simulink model "Twin_Builder"  (R2026a)
settings: Solver=VariableStepAuto  StopTime=simTime  FixedStep=Ts/60  RelTol=1e-2
values from neighbouring files (symbols this model uses):
  ac = log(9)/tr    [Run_Twin.m]
  as = 0.08 * ac    [Run_Twin.m]
  ath = 0.25 * as    [Run_Twin.m]
  B = 0.00001    (= 1e-05)    [Run_Twin.m]
  BEMFD_FEA_PerHz = InterpFEA_Data_ForSimulink(FEA_Data.BackEMFD_perHz, IS_FEA, IEA_FEA, IS_Interp, IEA_Interp)    [Run_Twin.m]
  BEMFQ_FEA_PerHz = InterpFEA_Data_ForSimulink(FEA_Data.BackEMFQ_perHz, IS_FEA, IEA_FEA, IS_Interp, IEA_Interp)    [Run_Twin.m]
  CondLoss_Inv = zeros([length(IS_Interp), size(FEA_Data.ConductionLoss, [2 3] ) ])    [Run_Twin.m]
  CopperLoss_FEA = InterpFEA_Data_ForSimulink(FEA_Data.CopperLosses, IS_FEA, IEA_FEA, IS_Interp, IEA_Interp)    [Run_Twin.m]
  DriveMethod = 1    [Run_Twin.m]
  EnvTorque_FW = interp1(Speed_full, Env_full, Speed_Vec, 'pchip', 'extrap')    [Run_Twin.m]
  f_sw = 10e3    (= 10000)    [Run_Twin.m]
  FEA_Data = LoadData.(FieldData{1})    [Run_Twin.m]
  FILTER_COEFF = 0.23    [Run_Twin.m]
  FluxD_FEA = InterpFEA_Data_ForSimulink(FEA_Data.FluxD, IS_FEA, IEA_FEA, IS_Interp, IEA_Interp)    [Run_Twin.m]
  FluxQ_FEA = InterpFEA_Data_ForSimulink(FEA_Data.FluxQ, IS_FEA, IEA_FEA, IS_Interp, IEA_Interp)    [Run_Twin.m]
  FrictLoss_FEA = squeeze( FEA_Data.FrictLosses(1,1,:) )    [Run_Twin.m]
  GateLoss_Inv = zeros([length(IS_Interp), size(FEA_Data.ConductionLoss, [2 3] ) ])    [Run_Twin.m]
  IDcore_FEA = InterpFEA_Data_ForSimulink(FEA_Data.IDc, IS_FEA, IEA_FEA, IS_Interp, IEA_Interp)    [Run_Twin.m]
  IEA_FEA = IEA_Interp    [Run_Twin.m]
  IQcore_FEA = InterpFEA_Data_ForSimulink(FEA_Data.IQc, IS_FEA, IEA_FEA, IS_Interp, IEA_Interp)    [Run_Twin.m]
  IronLoss_FEA = InterpFEA_Data_ForSimulink(FEA_Data.IronLosses,   IS_FEA, IEA_FEA, IS_Interp, IEA_Interp)    [Run_Twin.m]
  Is_Amp = 40    [Run_Twin.m]
  IS_FEA = IS_Interp    [Run_Twin.m]
  J = FEA_Data.Jinertia    [Run_Twin.m]
  J_Control = FEA_Data.Jinertia    [Run_Twin.m]
  LD_FEA = InterpFEA_Data_ForSimulink(FEA_Data.LD, IS_FEA, IEA_FEA, IS_Interp, IEA_Interp)    [Run_Twin.m]
  LD_Single = mean(LD_FEA, 'all')    [Run_Twin.m]
  LQ_FEA = InterpFEA_Data_ForSimulink(FEA_Data.LQ, IS_FEA, IEA_FEA, IS_Interp, IEA_Interp)    [Run_Twin.m]
  LQ_Single = mean(LQ_FEA, 'all')    [Run_Twin.m]
  MagnetLoss_FEA = InterpFEA_Data_ForSimulink(FEA_Data.MagnetLosses, IS_FEA, IEA_FEA, IS_Interp, IEA_Interp)    [Run_Twin.m]
  MaxSpeed = max(Speed_Vec)    [Run_Twin.m]
  MaxTe = max(Torque_FEA, [], 'all')    [Run_Twin.m]
  ModStrategy = 1    [Run_Twin.m]
  PMFlux_FEA = interp1(IS_FEA, squeeze( FEA_Data.FluxD(:,IEA_FEA == 90, :) ), IS_Interp, 'pchip' )    [Run_Twin.m]
  PMFlux_Single = mean( PMFlux_FEA, 'all' )    [Run_Twin.m]
  PMT_ID = round( F_ID(PMT_grid, Speed_grid), 2)    [Run_Twin.m]
  PMT_IQ = round( F_IQ(PMT_grid, Speed_grid), 2)    [Run_Twin.m]
  PMT_Vec = linspace(0,   100,   InterpSamples)    [Run_Twin.m]
  PolePair = FEA_Data.Poles / 2    [Run_Twin.m]
  PPR = 1024    [Run_Twin.m]
  ProxiLoss_FEA = InterpFEA_Data_ForSimulink(FEA_Data.ProxiLosses,  IS_FEA, IEA_FEA, IS_Interp, IEA_Interp)    [Run_Twin.m]
  Rcore_FEA = InterpFEA_Data_ForSimulink(FEA_Data.Rcore, IS_FEA, IEA_FEA, IS_Interp, IEA_Interp)    [Run_Twin.m]
  RDC = squeeze( Rseries_FEA(1,1,1) )    [Run_Twin.m]
  RefSpeed = [50, 400, 250, 500, 400]    [Run_Twin.m]
  RefTheta = [50, 0, 140, 300, -50]    [Run_Twin.m]
  Rseries_FEA = InterpFEA_Data_ForSimulink(FEA_Data.Rs,    IS_FEA, IEA_FEA, IS_Interp, IEA_Interp)    [Run_Twin.m]
  ShafthLoad = [10, 25, 3, 8, 10]    [Run_Twin.m]
  simTime = mechThetaTarget / wMechTarget    [Run_Twin.m]
  Speed_FEA = FEA_Data.Speed_vec    [Run_Twin.m]
  Speed_Vec = linspace(min(Speed_full), max(Speed_full), InterpSamples)    [Run_Twin.m]
  speedTarget = 200    [Run_Twin.m]
  SR_FEA = FEA_Data.SynchAngle    [Run_Twin.m]
  SwitchLoss_Inv = zeros([length(IS_Interp), size(FEA_Data.ConductionLoss, [2 3] ) ])    [Run_Twin.m]
  Tdt = 0.3 * 1e-6    (= 3e-07)    [Run_Twin.m]
  Throttle = 45    [Run_Twin.m]
  Times = [0, 0.2, 0.4, 0.6, 0.8] * simTime    [Run_Twin.m]
  Torque_FEA = InterpFEA_Data_ForSimulink(FEA_Data.TorqueFEA, IS_FEA, IEA_FEA, IS_Interp, IEA_Interp)    [Run_Twin.m]
  Ts = 1/f_sw    (= 0.0001)    [Run_Twin.m]
  Ts_Sp = 2 * Ts    (= 0.0002)    [Run_Twin.m]
  Vdc = 56    [Run_Twin.m]
  Vs_pu = 0.98    [Run_Twin.m]
  WindageLoss_FEA = squeeze( FEA_Data.WindLosses(1,1,:) )    [Run_Twin.m]
undefined symbols (not defined in the file or in its folder): DiscIntNeverNeededParam, feNom, mf, OverMod, PMT_Speed, SimData, Tables
libraries: simulink x14, ee_lib x11, simulink_extras x7, eeTransforms x6, fl_lib x6, eeGeneralControl x4, spsMeanLib x2, dspxfrm3 x1
(part 1 of 3)
settings Model: Creator=antho  LastModifiedBy=antho
settings SolverCC: ZeroCrossAlgorithm=Adaptive
settings DebuggingCC: ArtificialAlgebraicLoopMsg=none  MaskedZcDiagnostic=none  IgnoredZcDiagnostic=none
settings SimscapeCC: SimscapeNominalValues="[{\"value\":\"1\",\"unit\":\"A\"},{\"value\":\"1\",\"unit\":\"bar\"},{\"value\":\"1\",\"unit\":\"cm^2\"},{\"value\":\"1\",\"unit\":\"cm^3/s\"},{\"value\":\"1\",\"unit\":\"kJ/kg\"},{\"value\":\"1\",\"unit\":\"kW\"},{\"value\":\"1\",\"unit\":\"l\"},{\"value\":\"1\",\"unit\":\"N\"},{\"value\":\"1\",\"unit\":\"N*m\"},{\"value\":\"1\",\"unit\":\"V\"}]"  SimscapeLogType=none  SimscapeLogDataHistory=5000.0

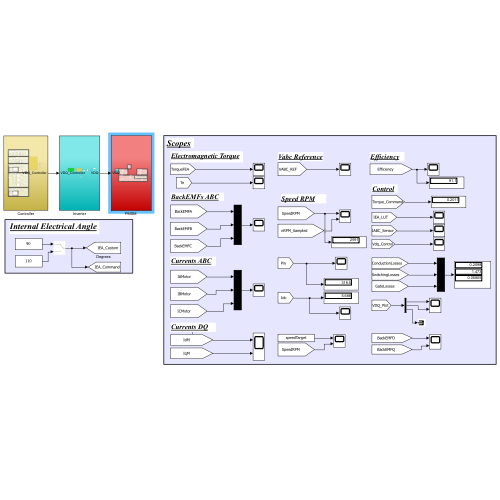
[thumbnail: Simulink's stored preview of the top-level diagram]
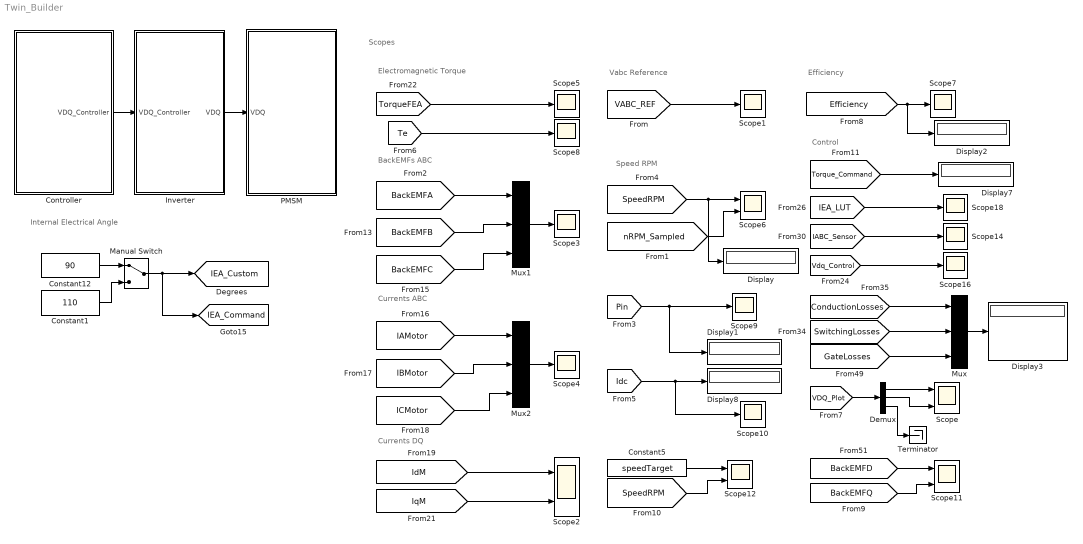
== system Twin_Builder ==
  note: Currents ABC
  note: BackEMFs ABC
  note: Scopes
  note: Electromagnetic Torque
  note: Currents DQ
  note: Vabc Reference
  note: Speed RPM
  note: Internal Electrical Angle
  note: Efficiency
  note: Control
  Constant1 : Constant  Value=110  VectorParams1D=off  SampleTime=0
  Constant12 : Constant  Value=90  VectorParams1D=off  SampleTime=0
  Constant5 : Constant  Value=speedTarget  SampleTime=Ts
  Controller : Subsystem
  Demux : Demux  Outputs=3
  Display{,1..3,7..8} (6 alike) : Display
  Inverter : Subsystem
  Manual Switch : ManualSwitch
  Mux : Mux  Inputs=3
  Mux1 : Mux  Inputs=3
  Mux2 : Mux  Inputs=3
  "PMSM " : Subsystem
  Scope{,2,6,11..12} (5 alike) : Scope  NumInputPorts=2
      Scope settings: ActiveDisplayYMinimum=-43.33518  ActiveDisplayYMaximum=40.81845
      Scope11 settings: ActiveDisplayYMinimum=-5.31808  ActiveDisplayYMaximum=1.44392  DataLoggingVariableName=ScopeData2
      Scope12 settings: ActiveDisplayYMinimum=1475.9301024865783  ActiveDisplayYMaximum=1516.335592593025  DataLoggingVariableName=ScopeData22
      Scope2 settings: ActiveDisplayYMinimum=-5.9549540447298286  ActiveDisplayYMaximum=6.9473157264243515  DataLoggingVariableName=ScopeData7
      Scope6 settings: ActiveDisplayYMinimum=-188.56958986761623  ActiveDisplayYMaximum=1697.1263088085464
  Scope{1,3..5,7..10,14,16,18} (11 alike) : Scope
      Scope1 settings: ActiveDisplayYMinimum=-0.12499999999999997  ActiveDisplayYMaximum=1.125
      Scope10 settings: ActiveDisplayYMinimum=-10.699535134143511  ActiveDisplayYMaximum=61.951701868549058
      Scope14 settings: ActiveDisplayYMinimum=-35.97658  ActiveDisplayYMaximum=53.42367
      Scope16 settings: ActiveDisplayYMinimum=-13.11859  ActiveDisplayYMaximum=37.37662  DataLoggingVariableName=ScopeData5
      Scope18 settings: ActiveDisplayYMinimum=26.32642  ActiveDisplayYMaximum=197.07481
      Scope3 settings: ActiveDisplayYMinimum=-28.0068607396772  ActiveDisplayYMaximum=28.009786105867875  DataLoggingVariableName=ScopeData25
      Scope4 settings: ActiveDisplayYMinimum=-10.513567775174659  ActiveDisplayYMaximum=10.513016915714479  DataLoggingVariableName=ScopeData3
      Scope5 settings: ActiveDisplayYMinimum=0.36126733092148122  ActiveDisplayYMaximum=0.991709204534436  DataLoggingVariableName=ScopeData2
      Scope7 settings: ActiveDisplayYMinimum=90.703551699385159  ActiveDisplayYMaximum=92.220982491183165
      Scope8 settings: ActiveDisplayYMinimum=-8.4790158509726883  ActiveDisplayYMaximum=35.221572331501939  DataLoggingVariableName=ScopeData3
      Scope9 settings: ActiveDisplayYMinimum=-526.14083348977579  ActiveDisplayYMaximum=1930.1579846280983
  Terminator : Terminator
  tag scope: IEA_Command=global, IEA_Custom=global
  wires:
  [BackEMFB] -> Mux1/2
  [BackEMFA] -> Mux1/1
  [IqM] -> Scope2/2
  [BackEMFC] -> Mux1/3
  [IBMotor] -> Mux2/2
  Mux1/1 -> Scope3/1
  [ICMotor] -> Mux2/3
  Mux2/1 -> Scope4/1
  [IAMotor] -> Mux2/1
  [TorqueFEA] -> Scope5/1
  [IdM] -> Scope2/1
  [VABC_REF] -> Scope1/1
  [SpeedRPM] -> Scope6/1, Display/1
  Inverter/1(VDQ) -> "PMSM "/1(VDQ)
  [Te] -> Scope8/1
  [Efficiency] -> Display2/1, Scope7/1
  Controller/1(VDQ_Controller) -> Inverter/1(VDQ_Controller)
  [Torque_Command] -> Display7/1
  Constant12/1 -> Manual Switch/1
  Manual Switch/1 -> [IEA_Command], [IEA_Custom]
  Constant1/1 -> Manual Switch/2
  [Vdq_Control] -> Scope16/1
  [IEA_LUT] -> Scope18/1
  [IABC_Sensor] -> Scope14/1
  [nRPM_Sampled] -> Scope6/2
  [Pin] -> Display1/1, Scope9/1
  [GateLosses] -> Mux/3
  [SwitchingLosses] -> Mux/2
  [ConductionLosses] -> Mux/1
  Mux/1 -> Display3/1
  [Idc] -> Scope10/1, Display8/1
  Demux/3 -> Terminator/1
  Demux/2 -> Scope/2
  Demux/1 -> Scope/1
  [VDQ_Plot] -> Demux/1
  [BackEMFD] -> Scope11/1
  [BackEMFQ] -> Scope11/2
  Constant5/1 -> Scope12/1
  [SpeedRPM] -> Scope12/2

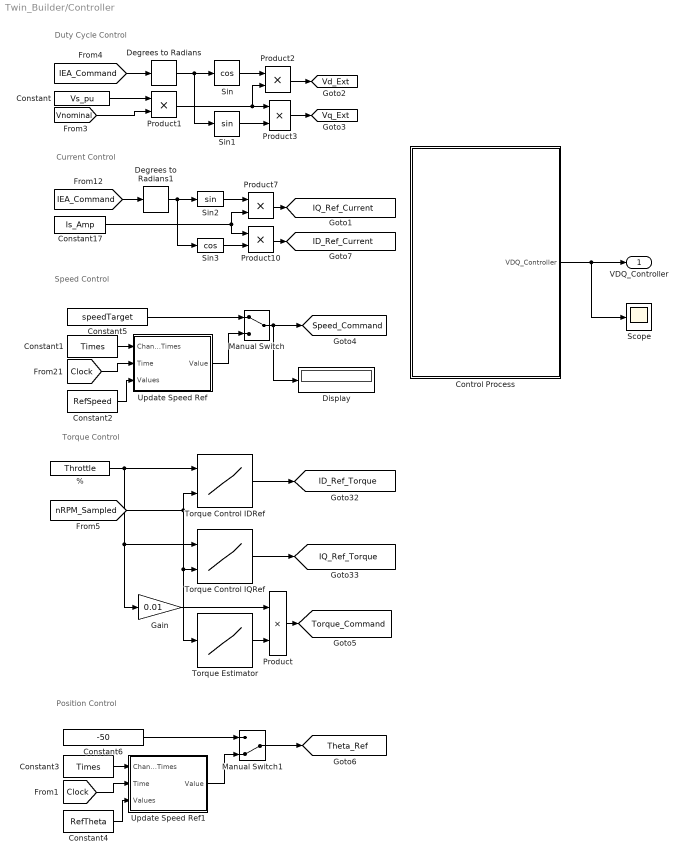
== system Twin_Builder/Controller ==
  note: Duty Cycle Control
  note: Speed Control
  note: Current Control
  note: Torque Control
  note: Position Control
  % : Constant  Value=Throttle  VectorParams1D=off  SampleTime=0
  Constant : Constant  Value=Vs_pu  SampleTime=0
  Constant1 : Constant  Value=Times
  Constant17 : Constant  Value=Is_Amp  SampleTime=0
  Constant2 : Constant  Value=RefSpeed
  Constant3 : Constant  Value=Times
  Constant4 : Constant  Value=RefTheta
  Constant5 : Constant  Value=speedTarget  SampleTime=Ts
  Constant6 : Constant  Value=-50  SampleTime=Ts
  Control Process : Subsystem
  Degrees to Radians : simulink_extras/Transformations/Degrees to Radians
  Degrees to Radians1 : simulink_extras/Transformations/Degrees to Radians
  Display : Display
  Gain : Gain  Gain=0.01
  Manual Switch : ManualSwitch
  Manual Switch1 : ManualSwitch  CurrentSetting=0
  Product{,1..3,7,10} (6 alike) : Product
  Scope : Scope
      settings: ActiveDisplayYMinimum=-9.29519  ActiveDisplayYMaximum=32.08868  DataLoggingVariableName=ScopeData2
  Sin : Trigonometry  Operator=cos
  Sin1 : Trigonometry
  Sin2 : Trigonometry
  Sin3 : Trigonometry  Operator=cos
  Torque Control IDRef : Lookup_n-D  BreakpointsForDimension1=PMT_Vec  BreakpointsForDimension2=Speed_Vec  Table=PMT_ID  InternalRulePriority=Speed  RndMeth=Simplest
      settings: InputPortMap=u0,u1
  Torque Control IQRef : Lookup_n-D  BreakpointsForDimension1=PMT_Vec  BreakpointsForDimension2=Speed_Vec  Table=PMT_IQ  InternalRulePriority=Speed  RndMeth=Simplest
      settings: InputPortMap=u0,u1
  Torque Estimator : Lookup_n-D  NumberOfTableDimensions=1  BreakpointsForDimension1=Speed_Vec  BreakpointsForDimension2=PMT_Speed(1,:)  Table=EnvTorque_FW  InternalRulePriority=Speed  RndMeth=Simplest
  Update Speed Ref : MATLAB Function  TreatAsAtomicUnit=on
  Update Speed Ref1 : MATLAB Function  TreatAsAtomicUnit=on
  VDQ_Controller : Outport
  tag scope: ID_Ref_Current=global, ID_Ref_Torque=global, IQ_Ref_Current=global, IQ_Ref_Torque=global, Speed_Command=global, Theta_Ref=global, Torque_Command=global, Vd_Ext=global, Vq_Ext=global
  wires:
  Product2/1 -> [Vd_Ext]
  Product3/1 -> [Vq_Ext]
  Product1/1 -> Product2/2, Product3/1
  Degrees to Radians/1 -> Sin/1, Sin1/1
  Sin1/1 -> Product3/2
  Sin/1 -> Product2/1
  [IEA_Command] -> Degrees to Radians/1
  Constant/1 -> Product1/1
  [Vnominal] -> Product1/2
  Product7/1 -> [IQ_Ref_Current]
  Degrees to Radians1/1 -> Sin3/1, Sin2/1
  Sin2/1 -> Product7/1
  Product10/1 -> [ID_Ref_Current]
  [IEA_Command] -> Degrees to Radians1/1
  Constant17/1 -> Product10/1, Product7/2
  Sin3/1 -> Product10/2
  %/1 -> Torque Control IDRef/1, Torque Control IQRef/1, Gain/1
  Torque Control IQRef/1 -> [IQ_Ref_Torque]
  Torque Control IDRef/1 -> [ID_Ref_Torque]
  [nRPM_Sampled] -> Torque Estimator/1, Torque Control IQRef/2, Torque Control IDRef/2
  Product/1 -> [Torque_Command]
  Torque Estimator/1 -> Product/2
  Gain/1 -> Product/1
  Update Speed Ref/1(Value) -> Manual Switch/2
  Constant2/1 -> Update Speed Ref/3(Values)
  Constant1/1 -> Update Speed Ref/1(ChangeTimes)
  [Clock] -> Update Speed Ref/2(Time)
  Constant5/1 -> Manual Switch/1
  Manual Switch/1 -> Display/1, [Speed_Command]
  Control Process/1(VDQ_Controller) -> VDQ_Controller/1, Scope/1
  Constant3/1 -> Update Speed Ref1/1(ChangeTimes)
  Update Speed Ref1/1(Value) -> Manual Switch1/2
  [Clock] -> Update Speed Ref1/2(Time)
  Constant4/1 -> Update Speed Ref1/3(Values)
  Manual Switch1/1 -> [Theta_Ref]
  Constant6/1 -> Manual Switch1/1

== system Twin_Builder/Inverter ==
  VDQ_Controller : Inport
  Create VRef : Subsystem
  MCU Delay : Delay  Commented=on  DelayLength=1  SampleTime=1.5*Ts
  Manual Switch : ManualSwitch  CurrentSetting=0
  PowerSwitches : Subsystem
  VDQ : Outport
  tag scope: VDQ_Plot=global
  wires:
  VDQ_Controller/1 -> Create VRef/1(VDQ_Controller)
  Create VRef/1(Vabc_Ref) -> PowerSwitches/1(Vabc_Ref)
  PowerSwitches/1(Vdq0) -> Manual Switch/1
  Manual Switch/1 -> [VDQ_Plot], VDQ/1
  [Vdq_Control] -> Manual Switch/2

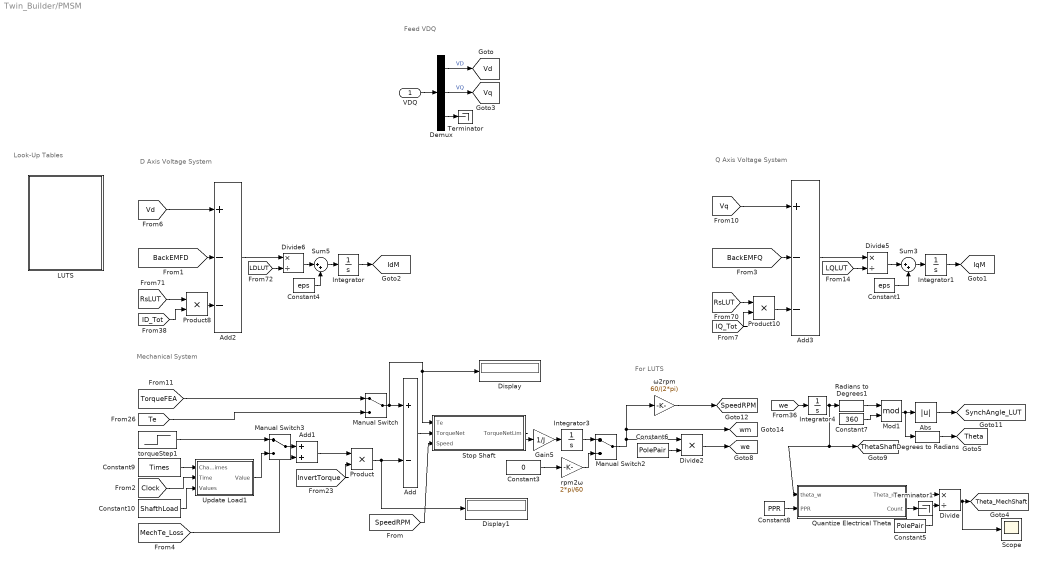
== system Twin_Builder/PMSM  ==
  note: Q Axis Voltage System
  note: D Axis Voltage System
  note: Feed VDQ
  note: Look-Up Tables
  note: Mechanical System
  note: For LUTS
  VDQ : Inport
  Abs : Abs  SaturateOnIntegerOverflow=off
  Add : Sum  Inputs=+-
  Add1 : Sum
  Add2 : Sum  Inputs=+--
  Add3 : Sum  Inputs=+--
  Constant1 : Constant  Value=eps  SampleTime=0
  Constant10 : Constant  Value=ShafthLoad
  Constant3 : Constant  Value=0  SampleTime=0
  Constant4 : Constant  Value=eps  SampleTime=0
  Constant5 : Constant  Value=PolePair
  Constant6 : Constant  Value=PolePair
  Constant7 : Constant  Value=360
  Constant8 : Constant  Value=PPR
  Constant9 : Constant  Value=Times
  Degrees to Radians : simulink_extras/Transformations/Degrees to Radians
  Demux : Demux  Outputs=3
  Display : Display
  Display1 : Display
  Divide : Product  Inputs=*/
  Divide2 : Product  Inputs=**
  Divide5 : Product  Inputs=*/
  Divide6 : Product  Inputs=*/
  Gain5 : Gain  Gain=1/J
  Integrator{,1,3..4} (4 alike) : Integrator
  LUTS : Subsystem
  Manual Switch : ManualSwitch
  Manual Switch2 : ManualSwitch
  Manual Switch3 : ManualSwitch
  Mod1 : Math  Operator=mod
  Product : Product
  Product10 : Product
  Product8 : Product
  "Quantize Electrical Theta " : MATLAB Function  TreatAsAtomicUnit=on
  Radians to Degrees1 : simulink_extras/Transformations/Radians to Degrees
  Scope : Scope
      settings: ActiveDisplayYMinimum=6.6141363545978225  ActiveDisplayYMaximum=6.6434972553948457  DataLoggingVariableName=ScopeData31
  Stop Shaft : MATLAB Function  TreatAsAtomicUnit=on
  Sum3 : Sum  Inputs=|++
  Sum5 : Sum  Inputs=|++
  Terminator : Terminator
  Terminator1 : Terminator
  Update Load1 : MATLAB Function  TreatAsAtomicUnit=on
  rpm2ω : Gain  Gain=2*pi/60
  torqueStep1 : Step  Time=0  FinalValue=mechLoad  SampleTime=0
  ω2rpm : Gain  Gain=60/(2*pi)
  tag scope: IdM=global, IqM=global, SpeedRPM=global, SynchAngle_LUT=global, Theta=global, ThetaShaft=global, Theta_MechShaft=global, Vd=global, Vq=global, we=global, wm=global
  wires:
  [Vd] -> Add2/1
  [BackEMFQ] -> Add3/2
  Constant4/1 -> Sum5/2
  [LQLUT] -> Divide5/2
  [LDLUT] -> Divide6/2
  Divide6/1 -> Sum5/1
  Product10/1 -> Add3/3
  [IQ_Tot] -> Product10/2
  Product8/1 -> Add2/3
  Sum3/1 -> Integrator1/1
  [BackEMFD] -> Add2/2
  [ID_Tot] -> Product8/2
  Constant1/1 -> Sum3/2
  [RsLUT] -> Product8/1
  Sum5/1 -> Integrator/1
  [Vq] -> Add3/1
  Divide5/1 -> Sum3/1
  [RsLUT] -> Product10/1
  Add3/1 -> Divide5/1
  Add2/1 -> Divide6/1
  Demux/3 -> Terminator/1
  VDQ/1 -> Demux/1
  Demux/1 -> [Vd]  "VD"
  Demux/2 -> [Vq]  "VQ"
  Integrator/1 -> [IdM]
  Integrator1/1 -> [IqM]
  [Te] -> Manual Switch/2
  Gain5/1 -> Integrator3/1
  [TorqueFEA] -> Manual Switch/1
  Integrator4/1 -> "Quantize Electrical Theta "/1(theta_w), [ThetaShaft], Radians to Degrees1/1
  Constant7/1 -> Mod1/2
  Abs/1 -> [SynchAngle_LUT]
  ω2rpm/1 -> [SpeedRPM]
  Divide2/1 -> [we]
  Constant6/1 -> Divide2/2
  [we] -> Integrator4/1
  Radians to Degrees1/1 -> Mod1/1
  Mod1/1 -> Degrees to Radians/1, Abs/1
  Degrees to Radians/1 -> [Theta]
  [SpeedRPM] -> Stop Shaft/3(Speed)
  Add/1 -> Stop Shaft/2(TorqueNet)
  Stop Shaft/1(TorqueNetLim) -> Gain5/1
  Manual Switch/1 -> Display/1, Stop Shaft/1(Te), Add/1
  Integrator3/1 -> Manual Switch2/1
  Manual Switch2/1 -> Divide2/1, [wm], ω2rpm/1
  rpm2ω/1 -> Manual Switch2/2
  Constant3/1 -> rpm2ω/1
  Constant8/1 -> "Quantize Electrical Theta "/2(PPR)
  "Quantize Electrical Theta "/2(Count) -> Terminator1/1
  Constant5/1 -> Divide/2
  "Quantize Electrical Theta "/1(Theta_mcu) -> Divide/1
  Divide/1 -> Scope/1, [Theta_MechShaft]
  Constant9/1 -> Update Load1/1(ChangeTimes)
  Constant10/1 -> Update Load1/3(Values)
  [MechTe_Loss] -> Add1/2
  [Clock] -> Update Load1/2(Time)
  torqueStep1/1 -> Manual Switch3/1
  Update Load1/1(Value) -> Manual Switch3/2
  Manual Switch3/1 -> Add1/1
  [InvertTorque] -> Product/2
  Add1/1 -> Product/1
  Product/1 -> Display1/1, Add/2

== system Twin_Builder/Controller/Control Process ==
  Add2 : Sum
  Constant : Constant  Value=0
  Display2 : Display
  IDQ References from Speed Controller : Subsystem
  IDQ _Reference : Subsystem
  Mux : Mux  Inputs=2
  Speed Reference from Position Controller : Subsystem
  VDQ Reference from Current Controller Fundamental : Subsystem
  VDQ Reference from Voltage Controller : Subsystem
  Voltage Saturation : Subsystem
  VDQ_Controller : Outport
  wires:
  [ID_Ref] -> VDQ Reference from Current Controller Fundamental/1(ID_Ref)
  VDQ Reference from Current Controller Fundamental/1(VDQ_Current) -> Add2/1
  [Speed_Ref] -> IDQ References from Speed Controller/1(SpeedRef)
  [Vd_Ext] -> VDQ Reference from Voltage Controller/1(Vd_Ext)
  [Vq_Ext] -> VDQ Reference from Voltage Controller/2(Vq_Ext)
  VDQ Reference from Voltage Controller/1(VDQ_Voltage) -> Add2/2
  [IQ_Ref] -> Display2/1, VDQ Reference from Current Controller Fundamental/2("IQ_Ref ")
  [Theta_Ref] -> Speed Reference from Position Controller/1(Theta_Ref)
  Add2/1 -> Mux/1
  Constant/1 -> Mux/2
  Mux/1 -> VDQ_Controller/1

== system Twin_Builder/Inverter/Create VRef ==
  note: Vabc_Ref Generation
  VDQ_Controller : Inport
  Add2 : Sum
  Constant : Constant  Value=OverMod  SampleTime=0
  Determine Common Mode Signal : Subsystem
  Divide : Product  Inputs=**/
  Finalize References : Subsystem
  Inverse Park Transform : eeTransforms/Inverse Park Transform  AxisAlignment=D-axis  PowerInvariant=off
      settings: LibrarySourceBlock=|
      | ee_sl_lib/Mathematical
      | Transforms/Inverse
      | Park Transform
  Park Transform : eeTransforms/Park Transform  AxisAlignment=D-axis  PowerInvariant=off
      settings: LibrarySourceBlock=|
      | ee_sl_lib/Mathematical
      | Transforms/Park Transform
  Product : Product
  Product1 : Product
  Sample References : MATLAB Function  TreatAsAtomicUnit=on
  Scope : Scope
      settings: ActiveDisplayYMinimum=-0.125  ActiveDisplayYMaximum=1.125  DataLoggingVariableName=ScopeData4
  Vabc_Ref : Outport
  tag scope: VABC_REF=global, VDQ=global, Vabc_SPWM=global, Vdq_Control=global
  wires:
  [Theta_Sampled] -> Inverse Park Transform/2
  [CommonMode] -> Add2/2
  [Vnominal] -> Divide/3
  Constant/1 -> Divide/2
  [Overmod] -> Product/2
  [Vnominal] -> Product1/2
  Product1/1 -> [Vdq_Control]
  [Theta_Sampled] -> Park Transform/2
  Inverse Park Transform/1 -> Divide/1
  Add2/1 -> Product/1
  VDQ_Controller/1 -> [VDQ], Inverse Park Transform/1
  Divide/1 -> [Vabc_SPWM], Add2/1
  Finalize References/1(Vabc_Ref_Final) -> [VABC_REF], Scope/1, Vabc_Ref/1
  [Carrier] -> Sample References/2(TriSignal)
  Sample References/1(SampledSignals) -> Park Transform/1, Finalize References/1(Vabc_Ref)
  Product/1 -> Sample References/1(Signal)
  Park Transform/1 -> Product1/1

== system Twin_Builder/Inverter/PowerSwitches ==
  note: Inverter
  Vabc_Ref : Inport
  0.5 Ts PWM delay : Delay  DelayLength=1  SampleTime=Ts/2
  Add1 : Sum  Inputs=+-
  Cast To Boolean : DataTypeConversion  Commented=on  OutDataTypeStr=double  SaturateOnIntegerOverflow=off  RndMeth=Floor
  Cast To Boolean1 : DataTypeConversion  Commented=on  OutDataTypeStr=double  SaturateOnIntegerOverflow=off  RndMeth=Floor
  Cast To Boolean2 : DataTypeConversion  Commented=on  OutDataTypeStr=double  SaturateOnIntegerOverflow=off  RndMeth=Floor
  Cast To Boolean3 : DataTypeConversion  Commented=on  OutDataTypeStr=boolean  SaturateOnIntegerOverflow=off  RndMeth=Floor
  Cast To Boolean4 : DataTypeConversion  Commented=on  OutDataTypeStr=boolean  SaturateOnIntegerOverflow=off  RndMeth=Floor
  Cast To Boolean5 : DataTypeConversion  Commented=on  OutDataTypeStr=boolean  SaturateOnIntegerOverflow=off  RndMeth=Floor
  Constant2 : Constant  Value=Vdc  SampleTime=0
  Gain2 : Gain  Gain=1/3  RndMeth=Round  OutDataTypeStr=Inherit: Same as input
  Park Transform : eeTransforms/Park Transform  AxisAlignment=D-axis  PowerInvariant=off
      settings: LibrarySourceBlock=|
      | ee_sl_lib/Mathematical
      | Transforms/Park Transform
  Product1 : Product
  Relational Operator3 : RelationalOperator  OutDataTypeStr=boolean  RndMeth=Simplest  InputSameDT=off
  Scope1 : Scope
      settings: ActiveDisplayYMinimum=-40  ActiveDisplayYMaximum=40  DataLoggingVariableName=ScopeData2
  Sum of Elements : Sum  Inputs=+
  Transport Delay1 : TransportDelay  Commented=on  DelayTime=Tdt  TransDelayFeedthrough=on
  Transport Delay2 : TransportDelay  Commented=on  DelayTime=Tdt
  Transport Delay3 : TransportDelay  Commented=on  DelayTime=Tdt
  Vdq0 : Outport
  tag scope: VabcInv=global
  wires:
  Cast To Boolean1/1 -> Transport Delay2/1
  Cast To Boolean/1 -> Transport Delay1/1
  Transport Delay3/1 -> Cast To Boolean5/1
  Transport Delay2/1 -> Cast To Boolean4/1
  Transport Delay1/1 -> Cast To Boolean3/1
  Cast To Boolean2/1 -> Transport Delay3/1
  Vabc_Ref/1 -> 0.5 Ts PWM delay/1
  [Carrier] -> Relational Operator3/2
  Constant2/1 -> Product1/2
  Sum of Elements/1 -> Gain2/1
  Gain2/1 -> Add1/2
  Product1/1 -> Sum of Elements/1, Add1/1
  Add1/1 -> Park Transform/1, [VabcInv], Scope1/1
  [Theta] -> Park Transform/2
  Park Transform/1 -> Vdq0/1
  Relational Operator3/1 -> Product1/1
  0.5 Ts PWM delay/1 -> Relational Operator3/1

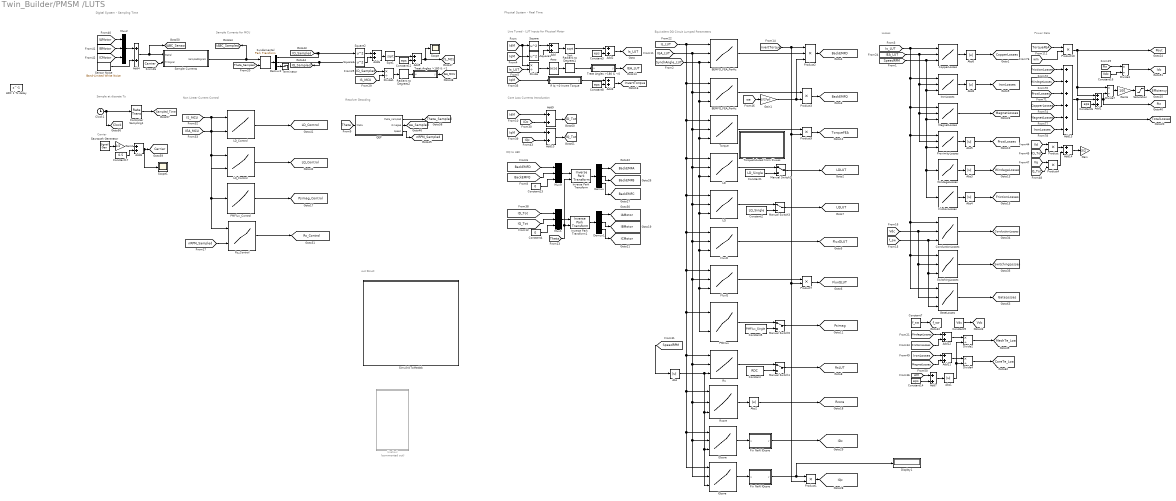
== system Twin_Builder/PMSM /LUTS ==
  note: out Struct
  note: Power Data
  note: Losses
  note: Equivalent DQ Circuit Lumped Parameters
  note: DQ to ABC
  note: Live Tuned - LUT Inputs for Physical Motor
  note: Physical System - Real Time
  note: Sample at discrete Ts
  note: Sample Currents for MCU
  note: Resolver Decoding
  note: Non Linear Current Control
  note: Digital System - Sampling Time
  note: Carrier
  note: Core Loss Currents Introduction
  ADC 1 Ts delay : Delay  DelayLength=1  SampleTime=Ts
  Abs{,1..6,8} (8 alike) : Abs  SaturateOnIntegerOverflow=off
  Acos : Trigonometry  Operator=acos  OutputSignalType=real
  Add{,2..12,14} (13 alike) : Sum
  Add1 : Sum  Inputs=+++
  Add13 : Sum  Inputs=++++++
  BEMFD_FEA_PerHz : Lookup_n-D  NumberOfTableDimensions=3  BreakpointsForDimension1=IS_FEA  BreakpointsForDimension2=IEA_FEA  BreakpointsForDimension3=SR_FEA  Table=BEMFD_FEA_PerHz  InternalRulePriority=Speed  RndMeth=Simplest
      settings: InputPortMap=u0,u1,u2
  BEMFQ_FEA_PerHz : Lookup_n-D  NumberOfTableDimensions=3  BreakpointsForDimension1=IS_FEA  BreakpointsForDimension2=IEA_FEA  BreakpointsForDimension3=SR_FEA  Table=BEMFQ_FEA_PerHz  InternalRulePriority=Speed  RndMeth=Simplest
      settings: InputPortMap=u0,u1,u2
  Clock1 : Clock
  ConductionLosses : Lookup_n-D  NumberOfTableDimensions=3  BreakpointsForDimension1=IS_FEA  BreakpointsForDimension2=FEA_Data.Vds_Vec  BreakpointsForDimension3=FEA_Data.fsw_Vec  BreakpointsForDimension4=FEA_Data.fsw_Vec  Table=CondLoss_Inv  InternalRulePriority=Speed  RndMeth=Simplest
      settings: InputPortMap=u0,u1,u2
  Constant : Constant  Value=RDC  SampleTime=0
  Constant1 : Constant  Value=LD_Single  SampleTime=0
  Constant{3,6,8,12} (4 alike) : Constant  Value=eps  SampleTime=0
  Constant13 : Constant  Value=0  SampleTime=0
  Constant14 : Constant  Value=eps
  Constant16 : Constant  Value=Vdc  SampleTime=0
  Constant17 : Constant  Value=0.5  SampleTime=0
  Constant2 : Constant  Value=LQ_Single  SampleTime=0
  Constant4 : Constant  Value=0  SampleTime=0
  Constant5 : Constant  Value=PMFlux_Single  SampleTime=0
  Constant7 : Constant  Value=f_sw  SampleTime=0
  Constant9 : Constant  Value=Vdc  SampleTime=0
  Controller Sampling1 : RateTransition  OutPortSampleTime=Ts
  CopperLosses : Lookup_n-D  NumberOfTableDimensions=3  BreakpointsForDimension1=IS_FEA  BreakpointsForDimension2=IEA_FEA  BreakpointsForDimension3=Speed_FEA  Table=CopperLoss_FEA  InternalRulePriority=Speed  RndMeth=Simplest
      settings: InputPortMap=u0,u1,u2
  Demux : Demux  Outputs=3
  Demux1 : Demux  Outputs=3
  Demux2 : Demux  Outputs=3
  Display1 : Display
  Divide{,1..4,7} (6 alike) : Product  Inputs=*/
  Fix NaN IDcore : MATLAB Function  TreatAsAtomicUnit=on
  Fix NaN IQcore : MATLAB Function  TreatAsAtomicUnit=on
  FluxD : Lookup_n-D  NumberOfTableDimensions=3  BreakpointsForDimension1=IS_FEA  BreakpointsForDimension2=IEA_FEA  BreakpointsForDimension3=SR_FEA  Table=FluxD_FEA  InternalRulePriority=Speed  RndMeth=Simplest
      settings: InputPortMap=u0,u1,u2
  FluxQ : Lookup_n-D  NumberOfTableDimensions=3  BreakpointsForDimension1=IS_FEA  BreakpointsForDimension2=IEA_FEA  BreakpointsForDimension3=SR_FEA  Table=FluxQ_FEA  InternalRulePriority=Speed  RndMeth=Simplest
      settings: InputPortMap=u0,u1,u2
  FrictionLosses : Lookup_n-D  NumberOfTableDimensions=1  BreakpointsForDimension1=Speed_FEA  BreakpointsForDimension2=SimData.IEA  BreakpointsForDimension3=SimData.speed_vec  Table=FrictLoss_FEA  InternalRulePriority=Speed  RndMeth=Simplest
  Fundamental : eeTransforms/Park Transform  AxisAlignment=D-axis  PowerInvariant=off
      settings: LibrarySourceBlock=|
      | ee_sl_lib/Mathematical
      | Transforms/Park Transform
  Gain : Gain  Gain=3/2
  Gain1 : Gain  Gain=1/(2*pi)
  Gain2 : Gain  Gain=1/2
  Gain6 : Gain  Gain=100
  "GateLosses " : Lookup_n-D  NumberOfTableDimensions=3  BreakpointsForDimension1=IS_FEA  BreakpointsForDimension2=FEA_Data.Vds_Vec  BreakpointsForDimension3=FEA_Data.fsw_Vec  BreakpointsForDimension4=FEA_Data.fsw_Vec  Table=GateLoss_Inv  InternalRulePriority=Speed  RndMeth=Simplest
      settings: InputPortMap=u0,u1,u2
  IDcore : Lookup_n-D  NumberOfTableDimensions=3  BreakpointsForDimension1=IS_FEA  BreakpointsForDimension2=IEA_FEA  BreakpointsForDimension3=Speed_FEA  Table=IDcore_FEA  InternalRulePriority=Speed  RndMeth=Simplest
      settings: InputPortMap=u0,u1,u2
  IQcore : Lookup_n-D  NumberOfTableDimensions=3  BreakpointsForDimension1=IS_FEA  BreakpointsForDimension2=IEA_FEA  BreakpointsForDimension3=Speed_FEA  Table=IQcore_FEA  InternalRulePriority=Speed  RndMeth=Simplest
      settings: InputPortMap=u0,u1,u2
  If Iq <0 Invert Torque : MATLAB Function  TreatAsAtomicUnit=on  SystemSampleTime=0
  Inverse Park Transform : eeTransforms/Inverse Park Transform  AxisAlignment=D-axis  PowerInvariant=off
      settings: LibrarySourceBlock=|
      | ee_sl_lib/Mathematical
      | Transforms/Inverse
      | Park Transform
  Inverse Park Transform1 : eeTransforms/Inverse Park Transform  AxisAlignment=D-axis  PowerInvariant=off
      settings: LibrarySourceBlock=|
      | ee_sl_lib/Mathematical
      | Transforms/Inverse
      | Park Transform
  IronLosses : Lookup_n-D  NumberOfTableDimensions=3  BreakpointsForDimension1=IS_FEA  BreakpointsForDimension2=IEA_FEA  BreakpointsForDimension3=Speed_FEA  Table=IronLoss_FEA  InternalRulePriority=Speed  RndMeth=Simplest
      settings: InputPortMap=u0,u1,u2
  LD : Lookup_n-D  NumberOfTableDimensions=3  BreakpointsForDimension1=IS_FEA  BreakpointsForDimension2=IEA_FEA  BreakpointsForDimension3=SR_FEA  Table=LD_FEA  InternalRulePriority=Speed  RndMeth=Simplest
      settings: InputPortMap=u0,u1,u2
  LD_Control : Lookup_n-D  BreakpointsForDimension1=FEA_Data.IS  BreakpointsForDimension2=FEA_Data.IEA  BreakpointsForDimension3=SimData.SynchAngle  Table=mean(FEA_Data.LD, 3)  InternalRulePriority=Speed  RndMeth=Simplest
      settings: InputPortMap=u0,u1
  LQ : Lookup_n-D  NumberOfTableDimensions=3  BreakpointsForDimension1=IS_FEA  BreakpointsForDimension2=IEA_FEA  BreakpointsForDimension3=SR_FEA  Table=LQ_FEA  InternalRulePriority=Speed  RndMeth=Simplest
      settings: InputPortMap=u0,u1,u2
  LQ_Control : Lookup_n-D  BreakpointsForDimension1=FEA_Data.IS  BreakpointsForDimension2=FEA_Data.IEA  BreakpointsForDimension3=SimData.SynchAngle  Table=mean(FEA_Data.LQ, 3)  InternalRulePriority=Speed  RndMeth=Simplest
      settings: InputPortMap=u0,u1
  MagnetLosses : Lookup_n-D  NumberOfTableDimensions=3  BreakpointsForDimension1=IS_FEA  BreakpointsForDimension2=IEA_FEA  BreakpointsForDimension3=Speed_FEA  Table=MagnetLoss_FEA  InternalRulePriority=Speed  RndMeth=Simplest
      settings: InputPortMap=u0,u1,u2
  Manual Switch{1..3,5} (4 alike) : ManualSwitch
  Mux1 : Mux  Inputs=3
  Mux2 : Mux  Inputs=3
  Mux9 : Mux  Inputs=3
  PMFlux : Lookup_n-D  BreakpointsForDimension1=IS_FEA  BreakpointsForDimension2=SR_FEA  BreakpointsForDimension3=Tables.Theta.Vectors.SychAngle  Table=PMFlux_FEA  InternalRulePriority=Speed  RndMeth=Simplest
      settings: InputPortMap=u0,u1
  PMFlux_Control : Lookup_n-D  NumberOfTableDimensions=1  BreakpointsForDimension1=FEA_Data.IS  BreakpointsForDimension2=SR_FEA  BreakpointsForDimension3=Tables.Theta.Vectors.SychAngle  Table="mean( squeeze( FEA_Data.FluxD(:, FEA_Data.IEA == 90, :)  ), 2)"  InternalRulePriority=Speed  RndMeth=Simplest
  Product{,1,3..4,7,9..10} (7 alike) : Product
  Product2 : Product  Inputs=3
  ProximityLosses : Lookup_n-D  NumberOfTableDimensions=3  BreakpointsForDimension1=IS_FEA  BreakpointsForDimension2=IEA_FEA  BreakpointsForDimension3=Speed_FEA  Table=ProxiLoss_FEA  InternalRulePriority=Speed  RndMeth=Simplest
      settings: InputPortMap=u0,u1,u2
  "QEP " : Subsystem
  Radians to Degrees1 : simulink_extras/Transformations/Radians to Degrees
  Radians to Degrees2 : simulink_extras/Transformations/Radians to Degrees
  Rcore : Lookup_n-D  NumberOfTableDimensions=3  BreakpointsForDimension1=IS_FEA  BreakpointsForDimension2=IEA_FEA  BreakpointsForDimension3=Speed_FEA  Table=Rcore_FEA  InternalRulePriority=Speed  RndMeth=Simplest
      settings: InputPortMap=u0,u1,u2
  Rs : Lookup_n-D  NumberOfTableDimensions=3  BreakpointsForDimension1=IS_FEA  BreakpointsForDimension2=IEA_FEA  BreakpointsForDimension3=Speed_FEA  Table=Rseries_FEA  InternalRulePriority=Speed  RndMeth=Simplest
      settings: InputPortMap=u0,u1,u2
  Rs_Control : Lookup_n-D  BreakpointsForDimension1=FEA_Data.IS  BreakpointsForDimension2=FEA_Data.Speed_vec  BreakpointsForDimension3=Speed_FEA  Table=squeeze( mean(FEA_Data.Rs, 2) )  InternalRulePriority=Speed  RndMeth=Simplest
      settings: InputPortMap=u0,u1
  Sample Currents : MATLAB Function  TreatAsAtomicUnit=on
  Saturation : Saturate  UpperLimit=100  LowerLimit=0
  Sawtooth Generator : SignalGenerator  WaveForm=sawtooth  Frequency=f_sw
  Scope : Scope
      settings: ActiveDisplayYMinimum=2.4366981448929863  ActiveDisplayYMaximum=9.594170017580808
  Scope1 : Scope
      settings: ActiveDisplayYMinimum=-0.12499999999999994  ActiveDisplayYMaximum=1.1249999999999998
  Sensor Noise : simulink/Sources/Band-Limited White Noise  Cov=[0.000001]  Ts=Ts  seed=[23341]
  SimulinkToMatlab : Subsystem
  Sqrt : Sqrt  OutputSignalType=real
  Sqrt1 : Sqrt
  Square{,1..3} (4 alike) : Math  Operator=square
  SwitchingLosses : Lookup_n-D  NumberOfTableDimensions=3  BreakpointsForDimension1=IS_FEA  BreakpointsForDimension2=FEA_Data.Vds_Vec  BreakpointsForDimension3=FEA_Data.fsw_Vec  BreakpointsForDimension4=FEA_Data.fsw_Vec  Table=SwitchLoss_Inv  InternalRulePriority=Speed  RndMeth=Simplest
      settings: InputPortMap=u0,u1,u2
  Terminator : Terminator
  Torque : Lookup_n-D  NumberOfTableDimensions=3  BreakpointsForDimension1=IS_FEA  BreakpointsForDimension2=IEA_FEA  BreakpointsForDimension3=SR_FEA  Table=Torque_FEA  InternalRulePriority=Speed  RndMeth=Simplest
      settings: InputPortMap=u0,u1,u2
  TorqueInduced from Fluxes : Subsystem
  Treat Angles >180 & <0 : MATLAB Function  TreatAsAtomicUnit=on
  Treat Angles >180 & <1 : MATLAB Function  TreatAsAtomicUnit=on
  Usefeul : Subsystem  Commented=on
  WindageLosses : Lookup_n-D  NumberOfTableDimensions=1  BreakpointsForDimension1=Speed_FEA  BreakpointsForDimension2=SimData.IEA  BreakpointsForDimension3=SimData.speed_vec  Table=WindageLoss_FEA  InternalRulePriority=Speed  RndMeth=Simplest
  tag scope: BackEMFA=global, BackEMFB=global, BackEMFC=global, BackEMFD=global, BackEMFQ=global, Carrier=global, Clock=global, ConductionLosses=global, CopperLosses=global, CoreTe_Loss=global, Efficiency=global, FluxDLUT=global, FluxQLUT=global, FrictionLosses=global, GateLosses=global, IABC_Sampled=global, IABC_Sensor=global, IAMotor=global, IBMotor=global, ICMotor=global, ID_Sampled=global, ID_Tot=global, IDc=global, IEA_LUT=global, IEA_MCU=global, IQ_Sampled=global, IQ_Tot=global, IQc=global, IS_MCU=global, Idc=global, InvertTorque=global, IronLosses=global, Is_LUT=global, LDLUT=global, LD_Control=global, LQLUT=global, LQ_Control=global, MagnetLosses=global, MechTe_Loss=global, Pin=global, Pout=global, ProxiLosses=global, Psimag=global, Psimag_Control=global, Rcore=global, RsLUT=global, Rs_Control=global, Sampled_Time=global, SwitchingLosses=global, Theta_Sampled=global, TorqueFEA=global, TotalLosses=global, Vdc=global, WindageLosses=global, f_sw=global, nRPM_Sampled=global, we_Sampled=global
  wires:
  [SynchAngle_LUT] -> BEMFD_FEA_PerHz/3, BEMFQ_FEA_PerHz/3, Torque/3, LD/3, LQ/3, FluxD/3, FluxQ/3, PMFlux/2
  [IqM] -> Square1/1
  [SpeedRPM] -> IronLosses/3, MagnetLosses/3, ProximityLosses/3, WindageLosses/1, FrictionLosses/1, CopperLosses/3
  Manual Switch3/1 -> [LQLUT]
  [Is_LUT] -> "GateLosses "/1, SwitchingLosses/1, ConductionLosses/1, ProximityLosses/1, MagnetLosses/1, IronLosses/1, CopperLosses/1
  Gain6/1 -> Saturation/1
  Sqrt/1 -> Add2/1
  Inverse Park Transform/1 -> Demux/1
  Rs/1 -> Manual Switch1/1
  [BackEMFQ] -> Mux9/2
  Inverse Park Transform1/1 -> Demux1/1
  Add2/1 -> [Is_LUT]
  Product7/1 -> [FluxQLUT]
  SwitchingLosses/1 -> [SwitchingLosses]
  Abs6/1 -> [CopperLosses]
  Constant9/1 -> [Vdc]
  Product9/1 -> [TorqueFEA]
  Demux/2 -> [BackEMFB]
  Constant4/1 -> Mux1/3
  Demux/3 -> [BackEMFC]
  Demux1/1 -> [IAMotor]
  Product3/1 -> [BackEMFQ]
  [IEA_LUT] -> ProximityLosses/2, MagnetLosses/2, IronLosses/2, CopperLosses/2
  [we] -> Gain1/1
  Add13/1 -> Add1/2, [TotalLosses]
  Demux1/3 -> [ICMotor]
  BEMFQ_FEA_PerHz/1 -> Product3/1
  [TorqueFEA] -> Product10/1
  [FrictionLosses] -> Add13/1
  [IqM] -> If Iq <0 Invert Torque/1(u)
  Abs8/1 -> [IronLosses]
  Rcore/1 -> Abs2/1
  Constant1/1 -> Manual Switch2/2
  ProximityLosses/1 -> Abs5/1
  [WindageLosses] -> Add13/2
  FrictionLosses/1 -> Abs4/1
  Square1/1 -> Add/2
  LD/1 -> Manual Switch2/1
  Square/1 -> Add/1
  Add1/1 -> Divide7/2, [Pin]
  Constant8/1 -> Add3/2
  FluxQ/1 -> Product7/1
  [MagnetLosses] -> Add13/5
  Constant5/1 -> Manual Switch5/2
  Manual Switch5/1 -> [Psimag]
  BEMFD_FEA_PerHz/1 -> Product2/2
  IronLosses/1 -> Abs8/1
  FluxD/1 -> [FluxDLUT]
  [InvertTorque] -> Product2/1, Product9/2, Product1/2, Product7/2
  Saturation/1 -> [Efficiency]
  Constant3/1 -> Add2/2
  Demux1/2 -> [IBMotor]
  CopperLosses/1 -> Abs6/1
  ConductionLosses/1 -> [ConductionLosses]
  [Is_LUT] -> Torque/1, LD/1, FluxQ/1, PMFlux/1, IDcore/1, IQcore/1, Rcore/1, Rs/1, FluxD/1, LQ/1, BEMFQ_FEA_PerHz/1, BEMFD_FEA_PerHz/1
  Constant7/1 -> [f_sw]
  Manual Switch1/1 -> [RsLUT]
  Divide3/1 -> [Idc]
  [IQ_Tot] -> Mux1/2
  WindageLosses/1 -> Abs3/1
  Gain1/1 -> Product3/2, Product2/3
  Mux9/1 -> Inverse Park Transform/1
  Divide/1 -> Acos/1
  Constant6/1 -> Add1/3
  Manual Switch2/1 -> [LDLUT]
  [IEA_LUT] -> BEMFD_FEA_PerHz/2, BEMFQ_FEA_PerHz/2, Torque/2, LD/2, LQ/2, FluxD/2, FluxQ/2, Rs/2, Rcore/2, IDcore/2, IQcore/2
  [IdM] -> Square/1, Divide/1
  Constant13/1 -> Mux9/3
  [IronLosses] -> Add13/6
  Radians to Degrees1/1 -> Treat Angles >180 & <0/1(u)
  [Pin] -> Divide3/1
  IQcore/1 -> Fix NaN IQcore/1(u)
  Product10/1 -> Divide7/1, Add1/1, [Pout]
  Torque/1 -> Product9/1
  Acos/1 -> Radians to Degrees1/1
  Constant16/1 -> Divide3/2
  Add/1 -> Sqrt/1
  LQ/1 -> Manual Switch3/1
  Abs5/1 -> [ProxiLosses]
  [SpeedRPM] -> Abs/1
  Divide7/1 -> Gain6/1
  If Iq <0 Invert Torque/1(y) -> Add3/1
  Fix NaN IDcore/1(y) -> [IDc]
  [ProxiLosses] -> Add13/3
  Constant2/1 -> Manual Switch3/2
  Abs4/1 -> [FrictionLosses]
  Treat Angles >180 & <0/1(y) -> [IEA_LUT]
  Demux/1 -> [BackEMFA]
  MagnetLosses/1 -> [MagnetLosses]
  [wm] -> Product10/2
  Abs2/1 -> [Rcore]
  PMFlux/1 -> Manual Switch5/1
  IDcore/1 -> Fix NaN IDcore/1(u)
  Product2/1 -> [BackEMFD]
  Constant/1 -> Manual Switch1/2
  Product1/1 -> [IQc]
  [ID_Tot] -> Mux1/1
  [Is_LUT] -> Divide/2
  [CopperLosses] -> Add13/4
  [BackEMFD] -> Mux9/1
  Abs3/1 -> [WindageLosses]
  Add3/1 -> [InvertTorque]
  [ICMotor] -> Mux2/3
  Controller Sampling1/1 -> [Sampled_Time]
  [IBMotor] -> Mux2/2
  Clock1/1 -> [Clock], Controller Sampling1/1
  Sensor Noise/1 -> Add4/2
  Add4/1 -> [IABC_Sensor], Sample Currents/1(Signal)
  Mux2/1 -> Add4/1
  Divide1/1 -> Radians to Degrees2/1
  Add5/1 -> Scope/1, [IS_MCU]
  Square3/1 -> Add6/2
  PMFlux_Control/1 -> [Psimag_Control]
  Rs_Control/1 -> [Rs_Control]
  Fundamental/1 -> Demux2/1
  [IAMotor] -> Mux2/1
  Demux2/3 -> Terminator/1
  Sqrt1/1 -> Add5/1
  Radians to Degrees2/1 -> Treat Angles >180 & <1/1(u)
  LD_Control/1 -> [LD_Control]
  Constant12/1 -> Add5/2
  Demux2/1 -> Square2/1, [ID_Sampled]
  [Carrier] -> Sample Currents/2(TriSignal)
  [IS_MCU] -> Rs_Control/1, PMFlux_Control/1, LQ_Control/1, LD_Control/1
  LQ_Control/1 -> [LQ_Control]
  [IEA_MCU] -> LD_Control/2, LQ_Control/2
  Treat Angles >180 & <1/1(y) -> [IEA_MCU]
  [Theta_Sampled] -> Fundamental/2
  Square2/1 -> Add6/1
  Demux2/2 -> Square3/1, [IQ_Sampled]
  [nRPM_Sampled] -> Rs_Control/2
  [ID_Sampled] -> Divide1/1
  Add6/1 -> Sqrt1/1
  [IS_MCU] -> Divide1/2
  "QEP "/1(theta_sampled) -> [Theta_Sampled]
  "QEP "/2(Omegae) -> [we_Sampled]
  "QEP "/3(Speed) -> [nRPM_Sampled]
  [Theta] -> "QEP "/1(theta)
  Constant17/1 -> Add8/2
  Gain2/1 -> Add8/1
  Sawtooth Generator/1 -> Gain2/1
  Add8/1 -> Scope1/1, [Carrier]
  [IDc] -> Add9/2
  [IdM] -> Add9/1
  [IQc] -> Add10/2
  [IqM] -> Add10/1
  Add9/1 -> [ID_Tot]
  Add10/1 -> [IQ_Tot]
  Fix NaN IQcore/1(y) -> Display1/1, Product1/1
  Add11/1 -> Divide4/1
  [MagnetLosses] -> Add11/2
  [IronLosses] -> Add11/1
  Add7/1 -> Abs1/1
  Constant14/1 -> Add7/2
  [wm] -> Add7/1
  Abs1/1 -> Divide2/2, Divide4/2
  Divide4/1 -> [CoreTe_Loss]
  [WindageLosses] -> Add12/1
  [FrictionLosses] -> Add12/2
  Add12/1 -> Divide2/1
  [Vdc] -> "GateLosses "/2, SwitchingLosses/2, ConductionLosses/2
  [f_sw] -> ConductionLosses/3, "GateLosses "/3, SwitchingLosses/3
  "GateLosses "/1 -> [GateLosses]
  [Vd] -> Product/1
  [ID_Tot] -> Product/2
  [Vq] -> Product4/1
  [IQ_Tot] -> Product4/2
  Product/1 -> Add14/1
  Product4/1 -> Add14/2
  Add14/1 -> Gain/1
  Mux1/1 -> Inverse Park Transform1/1
  [Theta] -> Inverse Park Transform1/2, Inverse Park Transform/2
  Sample Currents/1(SampledSignals) -> Fundamental/1, [IABC_Sampled]
  Abs/1 -> IQcore/3, IDcore/3, Rcore/3, Rs/3
  Divide2/1 -> [MechTe_Loss]

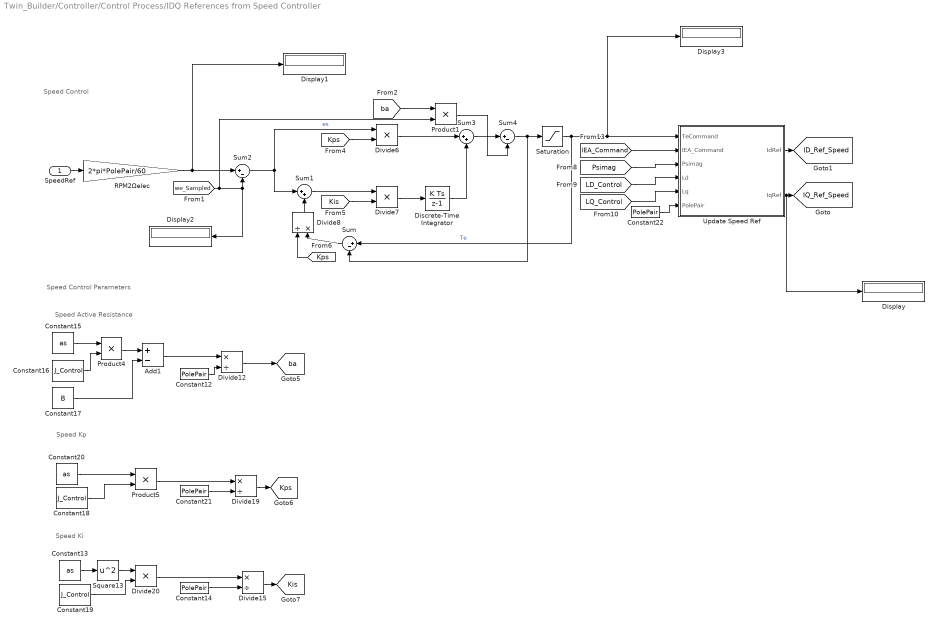
== system Twin_Builder/Controller/Control Process/IDQ References from Speed Controller ==
  note: Speed Control
  note: Speed Active Resistance
  note: Speed Kp
  note: Speed Control Parameters
  note: Speed Ki
  SpeedRef : Inport
  Add1 : Sum  Inputs=+-
  Constant{12,14,21..22} (4 alike) : Constant  Value=PolePair
  Constant13 : Constant  Value=as
  Constant15 : Constant  Value=as
  Constant16 : Constant  Value=J_Control
  Constant17 : Constant  Value=B
  Constant18 : Constant  Value=J_Control
  Constant19 : Constant  Value=J_Control
  Constant20 : Constant  Value=as
  Discrete-Time Integrator : DiscreteIntegrator  SampleTime=Ts  ICPrevOutput=DiscIntNeverNeededParam  ICPrevScaledInput=DiscIntNeverNeededParam
  Display{,1..3} (4 alike) : Display
  Divide12 : Product  Inputs=*/
  Divide15 : Product  Inputs=*/
  Divide19 : Product  Inputs=*/
  Divide20 : Product  Inputs=**
  Divide6 : Product  Inputs=**
  Divide7 : Product  Inputs=**
  Divide8 : Product  Inputs=/*
  Product1 : Product
  Product4 : Product
  Product5 : Product
  RPM2Ωelec : Gain  Gain=2*pi*PolePair/60
  Saturation : Saturate  UpperLimit=MaxTe  LowerLimit=-MaxTe
  Square13 : Math  Operator=square
  Sum : Sum  Inputs=|+-
  Sum1 : Sum  Inputs=|++
  Sum2 : Sum  Inputs=|+-
  Sum3 : Sum  Inputs=|++
  Sum4 : Sum  Inputs=|+-
  Update Speed Ref : MATLAB Function  TreatAsAtomicUnit=on
  tag scope: ID_Ref_Speed=global, IQ_Ref_Speed=global, Kis=global, Kps=global, ba=global
  wires:
  Sum2/1 -> Divide6/1, Sum1/1  "es"
  Sum3/1 -> Sum4/1
  Discrete-Time Integrator/1 -> Sum3/2
  Sum/1 -> Divide8/2
  Divide8/1 -> Sum1/2
  Sum1/1 -> Divide7/1
  [ba] -> Product1/1
  Product1/1 -> Sum4/2
  Sum4/1 -> Saturation/1, Sum/2
  [Kps] -> Divide6/2
  Divide6/1 -> Sum3/1
  [Kis] -> Divide7/2
  [Kps] -> Divide8/1
  Divide7/1 -> Discrete-Time Integrator/1
  RPM2Ωelec/1 -> Display1/1, Sum2/1
  [we_Sampled] -> Product1/2, Display2/1, Sum2/2
  Saturation/1 -> Display3/1, Update Speed Ref/1(TeCommand), Sum/1  "Te"
  SpeedRef/1 -> RPM2Ωelec/1
  Constant15/1 -> Product4/1
  Constant14/1 -> Divide15/2
  Constant16/1 -> Product4/2
  Constant17/1 -> Add1/2
  Divide20/1 -> Divide15/1
  Divide19/1 -> [Kps]
  Constant13/1 -> Square13/1
  Product4/1 -> Add1/1
  Divide15/1 -> [Kis]
  Constant21/1 -> Divide19/2
  Add1/1 -> Divide12/1
  Divide12/1 -> [ba]
  Constant12/1 -> Divide12/2
  Constant20/1 -> Product5/1
  Constant18/1 -> Product5/2
  Product5/1 -> Divide19/1
  Square13/1 -> Divide20/1
  Constant19/1 -> Divide20/2
  [IEA_Command] -> Update Speed Ref/2(IEA_Command)
  [Psimag] -> Update Speed Ref/3(Psimag)
  [LD_Control] -> Update Speed Ref/4(Ld)
  [LQ_Control] -> Update Speed Ref/5(Lq)
  Constant22/1 -> Update Speed Ref/6(PolePair)
  Update Speed Ref/1(IdRef) -> [ID_Ref_Speed]
  Update Speed Ref/2(IqRef) -> Display/1, [IQ_Ref_Speed]

== system Twin_Builder/Controller/Control Process/IDQ _Reference ==
  note: Determine Control Method
  Add : Sum
  Add1 : Sum
  Constant15 : Constant  Value=DriveMethod  SampleTime=0
  Demux : Demux  Outputs=2
  Determine Current Control : MATLAB Function  TreatAsAtomicUnit=on
  Determine Speed Control : MATLAB Function  TreatAsAtomicUnit=on
  Determine Torque Control : MATLAB Function  TreatAsAtomicUnit=on
  From2 : From  Commented=on  GotoTag=dIDQ  TagVisibility=global
  ID : Sum  Inputs=+++
  IQ : Sum  Inputs=+++
  Product{4..6,8..9,11} (6 alike) : Product
  tag scope: ID_Ref=global, IQ_Ref=global
  wires:
  Product4/1 -> ID/2
  Product11/1 -> IQ/2
  Product6/1 -> IQ/1
  [IQ_Ref_Torque] -> Product11/2
  [IQ_Ref_Speed] -> Product9/2
  Determine Torque Control/1(y) -> Product11/1, Product4/2
  Product8/1 -> ID/3
  Product5/1 -> ID/1
  Determine Current Control/1(y) -> Product6/1, Product5/2
  [ID_Ref_Torque] -> Product4/1
  Product9/1 -> IQ/3
  Constant15/1 -> Determine Speed Control/1(u), Determine Torque Control/1(u), Determine Current Control/1(u)
  Determine Speed Control/1(y) -> Product9/1, Product8/2
  [ID_Ref_Speed] -> Product8/1
  [IQ_Ref_Current] -> Product6/2
  [ID_Ref_Current] -> Product5/1
  ID/1 -> Add/1
  From2/1 -> Demux/1
  Add/1 -> [ID_Ref]
  Add1/1 -> [IQ_Ref]
  Demux/1 -> Add/2
  Demux/2 -> Add1/1
  IQ/1 -> Add1/2

== system Twin_Builder/Controller/Control Process/Speed Reference from Position Controller ==
  note: Position Control
  note: Speed Kp
  note: Position Control Parameters
  Theta_Ref : Inport
  Add : Sum
  Add7 : Sum  Inputs=+-
  Constant1 : Constant  Value=DriveMethod  SampleTime=0
  Constant20 : Constant  Value=ath
  Degrees to Radians : simulink_extras/Transformations/Degrees to Radians
  Determine Position Control : MATLAB Function  TreatAsAtomicUnit=on
  Determine Speed Control : MATLAB Function  TreatAsAtomicUnit=on
  Display : Display
  Product : Product  Inputs=3
  Product1 : Product
  Saturation : Saturate  UpperLimit=MaxSpeed  LowerLimit=-MaxSpeed
  Scope : Scope  NumInputPorts=2
      settings: ActiveDisplayYMinimum=-2.2103225046443447  ActiveDisplayYMaximum=6.3977065603751742  DataLoggingVariableName=ScopeData30
  rad/sTorpm : Gain  Gain=30/pi
  tag scope: Kpth=global, Speed_Ref=global
  wires:
  Theta_Ref/1 -> Degrees to Radians/1
  Degrees to Radians/1 -> Scope/1, Add7/1
  Add7/1 -> Product/1
  [Kpth] -> Product/2
  Constant1/1 -> Determine Position Control/1(u), Determine Speed Control/1(u)
  Determine Position Control/1(y) -> Product/3
  Determine Speed Control/1(y) -> Product1/1
  [Speed_Command] -> Product1/2
  Product1/1 -> Add/1
  Product/1 -> rad/sTorpm/1
  Add/1 -> Saturation/1
  Saturation/1 -> Display/1, [Speed_Ref]  "Speed RPM"
  rad/sTorpm/1 -> Add/2
  Constant20/1 -> [Kpth]
  [Theta_MechShaft] -> Scope/2, Add7/2

== system Twin_Builder/Controller/Control Process/VDQ Reference from Current Controller Fundamental ==
  ID_Ref : Inport
  "IQ_Ref " : Inport  Port=2
  Add : Sum  Inputs=+-
  Add1 : Sum  Inputs=+-
  Constant6 : Constant  Value=DriveMethod  SampleTime=0
  CurrentControlD : Subsystem
  CurrentControlQ : Subsystem
  Determine Control : MATLAB Function  TreatAsAtomicUnit=on
  Mux : Mux  Inputs=2
  Product : Product
  VDQ_Current : Outport
  tag scope: Error_D=global, Error_Q=global
  wires:
  Mux/1 -> Product/1
  Determine Control/1(y) -> Product/2
  Constant6/1 -> Determine Control/1(u)
  CurrentControlD/1(Vdref) -> Mux/1
  CurrentControlQ/1(Vqref) -> Mux/2
  Product/1 -> VDQ_Current/1
  Add/1 -> [Error_Q], CurrentControlQ/1(ErrorIq)
  [ID_Sampled] -> Add1/2
  ID_Ref/1 -> Add1/1
  Add1/1 -> [Error_D], CurrentControlD/1(ErrorId)
  [IQ_Sampled] -> Add/2
  "IQ_Ref "/1 -> Add/1

== system Twin_Builder/Controller/Control Process/VDQ Reference from Voltage Controller ==
  note: Voltage Control Parameters
  Vd_Ext : Inport
  Vq_Ext : Inport  Port=2
  Constant6 : Constant  Value=DriveMethod  SampleTime=0
  Determine Control : MATLAB Function  TreatAsAtomicUnit=on
  Divide1 : Product  Inputs=*/
  Divide2 : Product  Inputs=*/
  Mux1 : Mux  Inputs=2
  Product : Product
  Product1 : Product
  Product2 : Product
  VDQ_Voltage : Outport
  tag scope: VdExt_NoSat=global, VqExt_NoSat=global
  wires:
  [VMax_VoltControl] -> Divide1/2
  Vq_Ext/1 -> [VqExt_NoSat], Product1/1
  [Vnominal] -> Product/2
  Product2/1 -> VDQ_Voltage/1
  [Vnominal] -> Product1/2
  Product/1 -> Divide1/1
  [VMax_VoltControl] -> Divide2/2
  Product1/1 -> Divide2/1
  Vd_Ext/1 -> [VdExt_NoSat], Product/1
  Constant6/1 -> Determine Control/1(u)
  Mux1/1 -> Product2/1
  Determine Control/1(y) -> Product2/2
  Divide1/1 -> Mux1/1
  Divide2/1 -> Mux1/2

== system Twin_Builder/Controller/Control Process/Voltage Saturation ==
  note: Saturation
  Add : Sum  Inputs=+++
  Add1 : Sum  Inputs=+++
  Constant : Constant  Value=Vdc / 2  SampleTime=0
  Max : MinMax  Function=max  Inputs=2
  Max1 : MinMax  Function=max  Inputs=2
  Sqrt1 : Sqrt
  Sqrt3 : Sqrt
  Square{1..2,5..6} (4 alike) : Math  Operator=square
  Sum1 : Sum  Inputs=|++
  Sum3 : Sum  Inputs=|++
  tag scope: VMax_CurrControl=global, VMax_VoltControl=global, Vnominal=global
  wires:
  Square6/1 -> Sum3/2
  Square5/1 -> Sum3/1
  Sum3/1 -> Sqrt3/1
  Sqrt3/1 -> Max/1
  [Vnominal] -> Max/2
  Constant/1 -> [Vnominal]
  Max/1 -> [VMax_CurrControl]
  Max1/1 -> [VMax_VoltControl]
  Square1/1 -> Sum1/1
  [Vnominal] -> Max1/2
  Square2/1 -> Sum1/2
  Sqrt1/1 -> Max1/1
  Sum1/1 -> Sqrt1/1
  [Vd_NoSat] -> Add/1
  [Vd_12_NoSat] -> Add/3
  Add/1 -> Square5/1
  [Vq_NoSat] -> Add1/1
  [Vq_6_NoSat] -> Add1/2
  [Vq_12_NoSat] -> Add1/3
  Add1/1 -> Square6/1
  [Vd_Ext] -> Square1/1
  [Vq_Ext] -> Square2/1
  [Vd_6_NoSat] -> Add/2
